simulink model "lazo_traccion"  (R2026a)
settings: Solver=ode1  StopTime=PL.t_fin  FixedStep=1e-4
values from neighbouring files (symbols this model uses):
  K = V_dis/PT.ke    [parametros_traccion.m]    (also in simular_escenarios.m = KE; K.umbral = u; simular_traccion.m = KT; K.cuentas = P.cuentas)
undefined symbols (not defined in the file or in its folder): PL
settings Model: Creator=Mitsuki  LastModifiedBy=Mitsuki

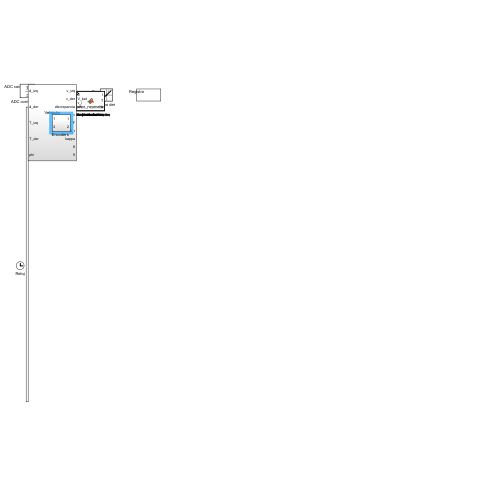
[thumbnail: Simulink's stored preview of the top-level diagram]
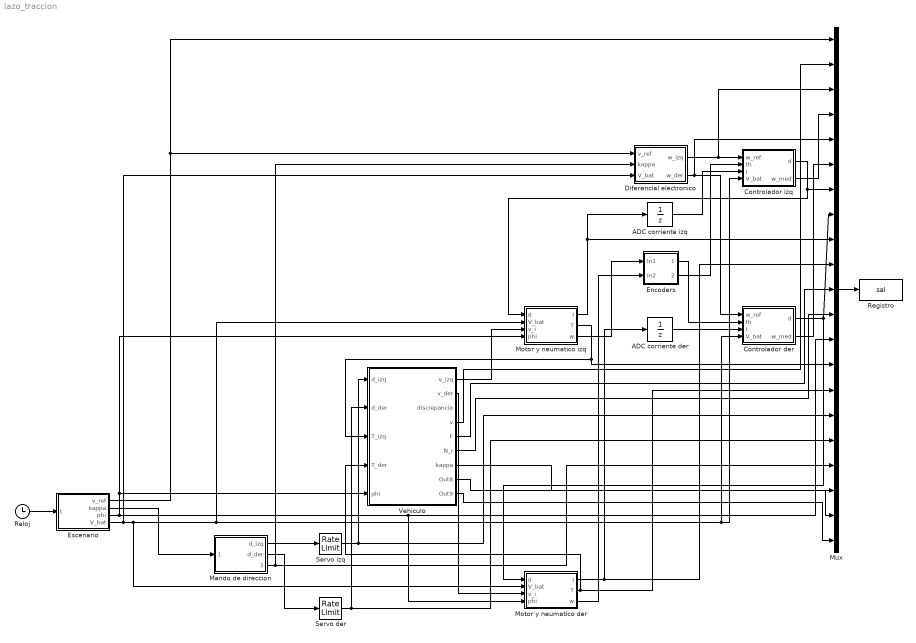
== system lazo_traccion ==
  ADC corriente der : UnitDelay  SampleTime=K.Ts
  ADC corriente izq : UnitDelay  SampleTime=K.Ts
  Controlador der : MATLAB Function  TreatAsAtomicUnit=on
  Controlador izq : MATLAB Function  TreatAsAtomicUnit=on
  Diferencial electronico : MATLAB Function  TreatAsAtomicUnit=on
  Encoders : Subsystem
  Escenario : MATLAB Function  TreatAsAtomicUnit=on
  Mando de direccion : MATLAB Function  TreatAsAtomicUnit=on
  Motor y neumatico der : MATLAB Function  TreatAsAtomicUnit=on
  Motor y neumatico izq : MATLAB Function  TreatAsAtomicUnit=on
  Mux : Mux  Inputs=21
  Registro : ToWorkspace  VariableName=sal  SampleTime=0.002
  Reloj : Clock
  Servo der : RateLimiter  RisingSlewLimit=PL.w_servo  FallingSlewLimit=-PL.w_servo  SampleTimeMode=inherited
  Servo izq : RateLimiter  RisingSlewLimit=PL.w_servo  FallingSlewLimit=-PL.w_servo  SampleTimeMode=inherited
  Vehiculo : Subsystem
  wires:
  Mando de direccion/2(d_der) -> Servo der/1
  Reloj/1 -> Escenario/1(t)
  Escenario/1(v_ref) -> Mux/1, Diferencial electronico/1(v_ref)
  Motor y neumatico izq/3(w) -> Encoders/1(In1)
  Mando de direccion/1(d_izq) -> Servo izq/1
  Diferencial electronico/2(w_der) -> Mux/5, Controlador der/1(w_ref)
  Escenario/2(kappa) -> Mando de direccion/1(kappa_ref)
  Escenario/3(phi) -> Motor y neumatico der/4(phi), Mux/13, Motor y neumatico izq/4(phi), Vehiculo/5(phi)
  Escenario/4(V_bat) -> Controlador izq/4(V_bat), Controlador der/4(V_bat), Motor y neumatico izq/2(V_bat), Motor y neumatico der/2(V_bat), Diferencial electronico/3(V_bat)
  Mando de direccion/3(kappa_fw) -> Diferencial electronico/2(kappa), Mux/18
  ADC corriente izq/1 -> Controlador izq/3(I)
  Vehiculo/5(F) -> Mux/11
  Servo izq/1 -> Vehiculo/1(d_izq), Mux/16
  Servo der/1 -> Mux/17, Vehiculo/2(d_der)
  Vehiculo/1(v_izq) -> Motor y neumatico izq/3(v_i)
  Motor y neumatico der/2(T) -> Vehiculo/4(T_der), Mux/15
  Vehiculo/2(v_der) -> Motor y neumatico der/3(v_i)
  Vehiculo/4(v) -> Mux/2
  Vehiculo/6(N_r) -> Mux/12
  Vehiculo/7(kappa) -> Mux/19
  Vehiculo/8(Out8) -> Mux/20
  ADC corriente der/1 -> Controlador der/3(I)
  Vehiculo/9(Out9) -> Mux/21
  Motor y neumatico izq/1(I) -> Mux/9, ADC corriente izq/1
  Motor y neumatico izq/2(T) -> Vehiculo/3(T_izq), Mux/14
  Mux/1 -> Registro/1
  Motor y neumatico der/1(I) -> Mux/10, ADC corriente der/1
  Motor y neumatico der/3(w) -> Encoders/2(In2)
  Diferencial electronico/1(w_izq) -> Mux/3, Controlador izq/1(w_ref)
  Encoders/1(Out1) -> Controlador der/2(th)
  Encoders/2(Out2) -> Controlador izq/2(th)
  Controlador der/1(d) -> Motor y neumatico der/1(d), Mux/8
  Controlador izq/1(d) -> Mux/7, Motor y neumatico izq/1(d)
  Controlador der/2(w_med) -> Mux/6
  Controlador izq/2(w_med) -> Mux/4

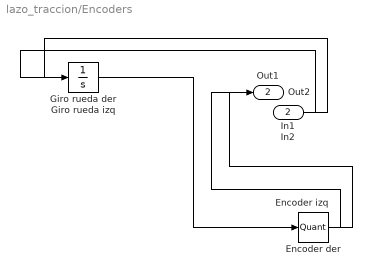
== system lazo_traccion/Encoders ==
  In1 : Inport
  In2 : Inport  Port=2
  Encoder der : Quantizer  QuantizationInterval=2*pi/PL.cuentas
  Encoder izq : Quantizer  QuantizationInterval=2*pi/PL.cuentas
  Giro rueda der : Integrator
  Giro rueda izq : Integrator
  Out1 : Outport
  Out2 : Outport  Port=2
  wires:
  Encoder izq/1 -> Out2/1
  Giro rueda izq/1 -> Encoder izq/1
  Giro rueda der/1 -> Encoder der/1
  Encoder der/1 -> Out1/1
  In1/1 -> Giro rueda izq/1
  In2/1 -> Giro rueda der/1

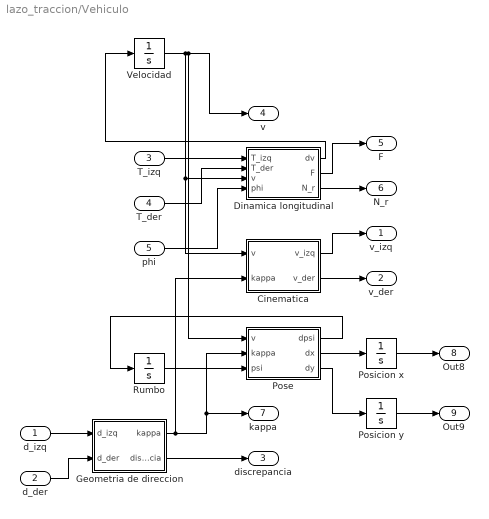
== system lazo_traccion/Vehiculo ==
  d_izq : Inport
  d_der : Inport  Port=2
  T_izq : Inport  Port=3
  T_der : Inport  Port=4
  phi : Inport  Port=5
  Cinematica : MATLAB Function  TreatAsAtomicUnit=on
  Dinamica longitudinal : MATLAB Function  TreatAsAtomicUnit=on
  Geometria de direccion : MATLAB Function  TreatAsAtomicUnit=on
  Pose : MATLAB Function  TreatAsAtomicUnit=on
  Posicion x : Integrator
  Posicion y : Integrator
  Rumbo : Integrator
  Velocidad : Integrator
  v_izq : Outport
  v_der : Outport  Port=2
  discrepancia : Outport  Port=3
  v : Outport  Port=4
  F : Outport  Port=5
  N_r : Outport  Port=6
  kappa : Outport  Port=7
  Out8 : Outport  Port=8
  Out9 : Outport  Port=9
  wires:
  phi/1 -> Dinamica longitudinal/4(phi)
  T_der/1 -> Dinamica longitudinal/2(T_der)
  T_izq/1 -> Dinamica longitudinal/1(T_izq)
  d_der/1 -> Geometria de direccion/2(d_der)
  d_izq/1 -> Geometria de direccion/1(d_izq)
  Velocidad/1 -> Dinamica longitudinal/3(v), Cinematica/1(v), Pose/1(v), v/1
  Rumbo/1 -> Pose/3(psi)
  Geometria de direccion/1(kappa) -> Pose/2(kappa), kappa/1, Cinematica/2(kappa)
  Geometria de direccion/2(discrepancia) -> discrepancia/1
  Dinamica longitudinal/1(dv) -> Velocidad/1
  Dinamica longitudinal/2(F) -> F/1
  Dinamica longitudinal/3(N_r) -> N_r/1
  Cinematica/1(v_izq) -> v_izq/1
  Cinematica/2(v_der) -> v_der/1
  Pose/1(dpsi) -> Rumbo/1
  Posicion y/1 -> Out9/1
  Pose/2(dx) -> Posicion x/1
  Posicion x/1 -> Out8/1
  Pose/3(dy) -> Posicion y/1

== matlab function lazo_traccion/Vehiculo/Cinematica ==
  data: v input; v_izq output; kappa input; v_der output; PL parameter
function [v_izq, v_der] = cinematica(v, kappa, PL)
% Velocidad del centro de cada rueda posterior (vía trasera PL.t)
v_izq = v*(1 - PL.t*kappa/2);
v_der = v*(1 + PL.t*kappa/2);

== matlab function lazo_traccion/Vehiculo/Dinamica longitudinal ==
  data: T_izq input; dv output; T_der input; v input; phi input; F output; N_r output; PL parameter
function [dv, F, N_r] = dinamica(T_izq, T_der, v, phi, PL)
% Equilibrio longitudinal de 505 con la masa de diseño
c = cosd(phi); s = sind(phi);
F = (T_izq + T_der)/PL.r;
F_rr = PL.fr*PL.m*PL.g*c*tanh(v/0.01);
dv = (F - PL.m*PL.g*s - F_rr)/(PL.m + 2*PL.J_rueda/PL.r^2);
N_f = (PL.m*PL.g*c*PL.Lcm - PL.m*PL.g*s*PL.hcm - PL.m*dv*PL.hcm)/PL.L;
N_r = PL.m*PL.g*c - N_f;

== matlab function lazo_traccion/Vehiculo/Pose ==
  data: v input; dpsi output; kappa input; psi input; dx output; dy output
function [dpsi, dx, dy] = pose(v, kappa, psi)
% Trayectoria del centro del eje posterior en el plano
dpsi = v*kappa;
dx = v*cos(psi);
dy = v*sin(psi);

== matlab function lazo_traccion/Mando de direccion ==
  settings: updateMethod=DISCRETE  sampleTime=K.Ts
  data: kappa_ref input; d_izq output; d_der output; kappa_fw output; K parameter
function [d_izq, d_der, kappa_fw] = mando_direccion(kappa_ref, K)
% Ackermann: ángulos de las ruedas frontales para la curvatura pedida, con la
% velocidad de cada consigna limitada a la del servo. kappa_fw es la curvatura que
% corresponde a esas consignas y la usa el diferencial electrónico.
persistent a_izq a_der
if isempty(a_izq), a_izq = 0; a_der = 0; end
kap = min(max(kappa_ref, -K.kappa_max), K.kappa_max);
obj_izq = atand(K.L*kap/(1 - K.b*kap/2));
obj_der = atand(K.L*kap/(1 + K.b*kap/2));
if K.w_servo > 0
    paso = K.w_servo*K.Ts;
    a_izq = a_izq + min(max(obj_izq - a_izq, -paso), paso);
    a_der = a_der + min(max(obj_der - a_der, -paso), paso);
else
    a_izq = obj_izq; a_der = obj_der;
end
d_izq = a_izq; d_der = a_der;
ti = tand(a_izq); td = tand(a_der);
kappa_fw = 0.5*(ti/(K.L + K.b*ti/2) + td/(K.L - K.b*td/2));

== matlab function lazo_traccion/Escenario ==
  data: t input; v_ref output; kappa output; phi output; V_bat output; PL parameter
function [v_ref, kappa, phi, V_bat] = escenario(t, PL)
% Velocidad en rampa de PL.a_ref hasta PL.v_nom; curvatura pedida por tramos
v_ref = min(PL.v_nom, PL.a_ref*max(0, t - PL.t_arr));
kappa = 0;
if t >= PL.giro(1) && t < PL.giro(2), kappa = PL.giro(3); end
if t >= PL.giro2(1) && t < PL.giro2(2), kappa = PL.giro2(3); end
phi = PL.pend0;
if t >= PL.pend_t(1), phi = PL.pend_t(2); end
V_bat = PL.V_bat;

== matlab function lazo_traccion/Diferencial electronico ==
  settings: updateMethod=DISCRETE  sampleTime=K.Ts
  data: v_ref input; w_izq output; kappa input; V_bat input; w_der output; K parameter; PL parameter
function [w_izq, w_der] = diferencial(v_ref, kappa, V_bat, K, PL)
% Velocidades de las ruedas posteriores para virar sin arrastre (505), con la vía trasera.
% Si la rueda exterior pediría más velocidad de la que el motor da con la tensión
% disponible, se reduce la velocidad de avance.
if K.limitar_curva > 0.5
    V_ef = min(K.V_mot, K.d_max_abs*V_bat);
    w_lim = (V_ef - K.R*K.I_plano)/K.ke;
    v_ref = min(v_ref, w_lim*K.r/(1 + K.t*abs(kappa)/2));
end
if PL.diferencial > 0.5
    w_izq = v_ref*(1 - K.t*kappa/2)/K.r;
    w_der = v_ref*(1 + K.t*kappa/2)/K.r;
else
    w_izq = v_ref/K.r; w_der = w_izq;
end

== matlab function lazo_traccion/Controlador izq ==
  settings: updateMethod=DISCRETE  sampleTime=K.Ts
  data: w_ref input; d output; th input; I input; V_bat input; w_med output; K parameter
function [d, w_med] = controlador_rueda(w_ref, th, I, V_bat, K)
% PI de velocidad de una rueda posterior (Arduino, cada K.Ts).
%   th: giro de la rueda contado por el encoder del motor [rad]; I: salida CS [A]
persistent th_ant xi
if isempty(th_ant), th_ant = th; xi = 0; end
w_med = (th - th_ant)/K.Ts;
th_ant = th;
e = w_ref - w_med;
d_max = min(K.d_max_abs, K.V_mot/V_bat);   % motor de 24 V con batería de hasta 29.4 V (603)
u = K.Kp*e + xi;
exceso = max(0, abs(I) - K.I_lim);          % límite de corriente de 8 A (603)
u = u - sign(u)*K.Kc*exceso;
d = min(max(u, -d_max), d_max);
if (abs(u) < d_max || sign(e) ~= sign(u)) && exceso == 0
    xi = xi + K.Ki*K.Ts*e;
end

== matlab function lazo_traccion/Controlador der ==
  settings: updateMethod=DISCRETE  sampleTime=K.Ts
  data: w_ref input; d output; th input; I input; V_bat input; w_med output; K parameter
function [d, w_med] = controlador_rueda(w_ref, th, I, V_bat, K)
% PI de velocidad de una rueda posterior (Arduino, cada K.Ts).
%   th: giro de la rueda contado por el encoder del motor [rad]; I: salida CS [A]
persistent th_ant xi
if isempty(th_ant), th_ant = th; xi = 0; end
w_med = (th - th_ant)/K.Ts;
th_ant = th;
e = w_ref - w_med;
d_max = min(K.d_max_abs, K.V_mot/V_bat);   % motor de 24 V con batería de hasta 29.4 V (603)
u = K.Kp*e + xi;
exceso = max(0, abs(I) - K.I_lim);          % límite de corriente de 8 A (603)
u = u - sign(u)*K.Kc*exceso;
d = min(max(u, -d_max), d_max);
if (abs(u) < d_max || sign(e) ~= sign(u)) && exceso == 0
    xi = xi + K.Ki*K.Ts*e;
end

== matlab function lazo_traccion/Motor y neumatico izq ==
  data: d input; I output; V_bat input; v_i input; phi input; T output; w output; PL parameter
function [I, T, w] = motor_neumatico(d, V_bat, v_i, phi, PL)
% Motorreductor con puente H (valores medios, sin inductancia) que mueve una
% rueda posterior con deslizamiento longitudinal lineal hasta mu·N.
c = cosd(phi); s = sind(phi);
N_r = PL.m*PL.g*c - (PL.m*PL.g*c*PL.Lcm - PL.m*PL.g*s*PL.hcm)/PL.L;
N_i = N_r/2;
F_max = PL.mu*N_i;
vr = max(abs(v_i), PL.v_min);
C = F_max/PL.s_pico;
a0 = PL.kt*(d*V_bat/PL.R - PL.I0*tanh(v_i/0.05));
a1 = PL.kt*PL.ke/PL.R;
w = (a0 + C*PL.r*v_i/vr)/(a1 + C*PL.r^2/vr);
F = C*(w*PL.r - v_i)/vr;
if abs(F) > F_max
    F = sign(F)*F_max;
    w = (a0 - F*PL.r)/a1;
end
I = (d*V_bat - PL.ke*w)/PL.R;
T = F*PL.r;

== matlab function lazo_traccion/Motor y neumatico der ==
  data: d input; I output; V_bat input; v_i input; phi input; T output; w output; PL parameter
function [I, T, w] = motor_neumatico(d, V_bat, v_i, phi, PL)
% Motorreductor con puente H (valores medios, sin inductancia) que mueve una
% rueda posterior con deslizamiento longitudinal lineal hasta mu·N.
c = cosd(phi); s = sind(phi);
N_r = PL.m*PL.g*c - (PL.m*PL.g*c*PL.Lcm - PL.m*PL.g*s*PL.hcm)/PL.L;
N_i = N_r/2;
F_max = PL.mu*N_i;
vr = max(abs(v_i), PL.v_min);
C = F_max/PL.s_pico;
a0 = PL.kt*(d*V_bat/PL.R - PL.I0*tanh(v_i/0.05));
a1 = PL.kt*PL.ke/PL.R;
w = (a0 + C*PL.r*v_i/vr)/(a1 + C*PL.r^2/vr);
F = C*(w*PL.r - v_i)/vr;
if abs(F) > F_max
    F = sign(F)*F_max;
    w = (a0 - F*PL.r)/a1;
end
I = (d*V_bat - PL.ke*w)/PL.R;
T = F*PL.r;

== matlab function lazo_traccion/Vehiculo/Geometria de direccion ==
  data: d_izq input; kappa output; d_der input; discrepancia output; PL parameter
function [kappa, discrepancia] = geometria(d_izq, d_der, PL)
% Curvatura que imponen los ángulos reales de las ruedas frontales. Si no cumplen
% Ackermann, cada rueda pide una curvatura distinta y la diferencia se arrastra.
ti = tand(d_izq); td = tand(d_der);
k_izq = ti/(PL.L + PL.b*ti/2);
k_der = td/(PL.L - PL.b*td/2);
kappa = 0.5*(k_izq + k_der);
discrepancia = k_izq - k_der;
